simulink model "Odometry"  (R2023b)
settings: Solver=FixedStepDiscrete  StartTime=0.0  StopTime=inf  FixedStep=t_sample_fast  RelTol=1e-3
settings Model: Creator=FIRSTMentor  LastModifiedBy=ander
settings OptimizationCC: DefaultParameterBehavior=Inlined  StrengthReduction=on  PassReuseOutputArgsAs=Individual arguments  ZeroExternalMemoryAtStartup=off  ZeroInternalMemoryAtStartup=off  OptimizeBlockOrder=speed  OptimizationPriority=Speed  OptimizationCustomize=off  MultiThreadedLoops=on  EfficientTunableParamExpr=on
settings DebuggingCC: MergeDetectMultiDrivingBlocksExec=none  ParameterTunabilityLossMsg=error
settings HardwareCC: ProdBitPerPointer=32  ProdBitPerSizeT=32  ProdBitPerPtrDiffT=32  ProdLargestAtomicInteger=Long  ProdWordSize=32  ProdHWDeviceType=ARM Compatible->ARM 7
settings ModelReferenceCC: PropagateSignalLabelsOutOfModel=off
settings SFSimCC: MATLABDynamicMemAlloc=off
settings RTWCC: Description=Embedded Coder  SystemTargetFile=ert.tlc  GenCodeOnly=on  TemplateMakefile=ert_default_tmf  Toolchain=MinGW64 | gmake (64-bit Windows)
settings CodeAppCC: ForceParamTrailComments=on  IgnoreCustomStorageClasses=off  OperatorAnnotations=on  SimulinkDataObjDesc=on  SFDataObjDesc=on  InsertBlockDesc=on
settings ERTTargetCC: TargetLangStandard=C99 (ISO)  UtilityFuncGeneration=Shared location  SupportVariableSizeSignals=on  ParenthesesLevel=Maximum  InlinedParameterPlacement=NonHierarchical  ERTCustomFileTemplate=example_file_process.tlc

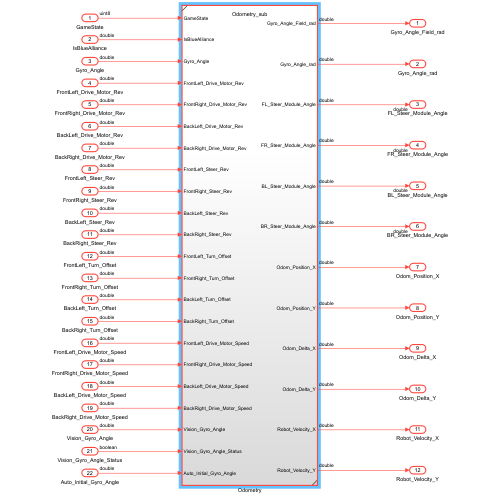
[thumbnail: Simulink's stored preview of the top-level diagram]
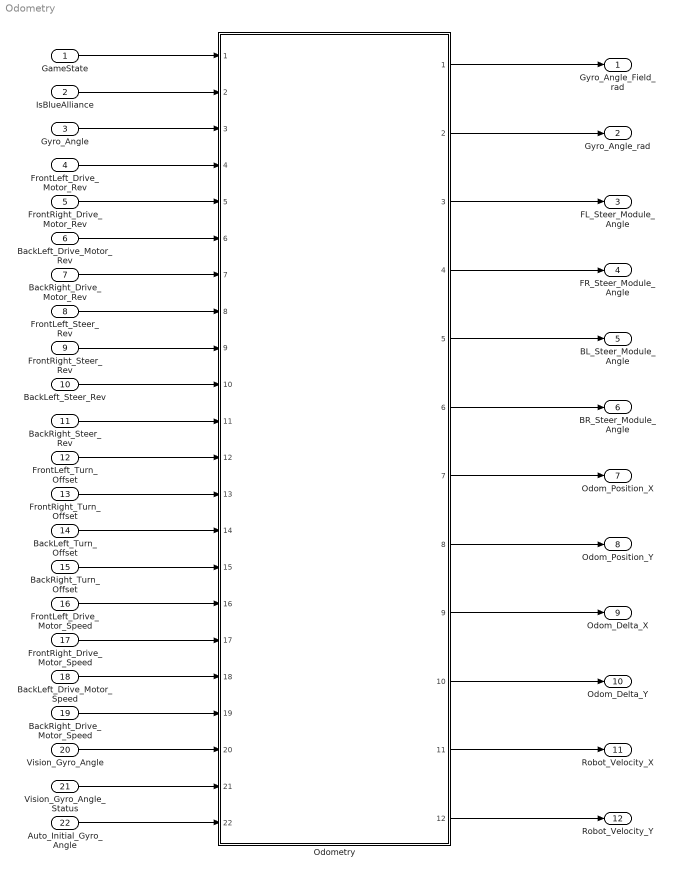
== system Odometry ==
  GameState : Inport
  IsBlueAlliance : Inport  Port=2
  Gyro_Angle : Inport  Port=3
  FrontLeft_Drive_Motor_Rev : Inport  Port=4
  FrontRight_Drive_Motor_Rev : Inport  Port=5
  BackLeft_Drive_Motor_Rev : Inport  Port=6
  BackRight_Drive_Motor_Rev : Inport  Port=7
  FrontLeft_Steer_Rev : Inport  Port=8
  FrontRight_Steer_Rev : Inport  Port=9
  BackLeft_Steer_Rev : Inport  Port=10
  BackRight_Steer_Rev : Inport  Port=11
  FrontLeft_Turn_Offset : Inport  Port=12
  FrontRight_Turn_Offset : Inport  Port=13
  BackLeft_Turn_Offset : Inport  Port=14
  BackRight_Turn_Offset : Inport  Port=15
  FrontLeft_Drive_Motor_Speed : Inport  Port=16
  FrontRight_Drive_Motor_Speed : Inport  Port=17
  BackLeft_Drive_Motor_Speed : Inport  Port=18
  BackRight_Drive_Motor_Speed : Inport  Port=19
  Vision_Gyro_Angle : Inport  Port=20
  Vision_Gyro_Angle_Status : Inport  Port=21
  Auto_Initial_Gyro_Angle : Inport  Port=22
  Odometry : Subsystem  ReferencedSubsystem=Odometry_sub
  Gyro_Angle_Field_rad : Outport
  Gyro_Angle_rad : Outport  Port=2
  FL_Steer_Module_Angle : Outport  Port=3  OutDataTypeStr=double  Unit=rad
  FR_Steer_Module_Angle : Outport  Port=4  OutDataTypeStr=double  Unit=rad
  BL_Steer_Module_Angle : Outport  Port=5  OutDataTypeStr=double  Unit=rad
  BR_Steer_Module_Angle : Outport  Port=6  OutDataTypeStr=double  Unit=rad
  Odom_Position_X : Outport  Port=7
  Odom_Position_Y : Outport  Port=8
  Odom_Delta_X : Outport  Port=9
  Odom_Delta_Y : Outport  Port=10
  Robot_Velocity_X : Outport  Port=11
  Robot_Velocity_Y : Outport  Port=12
  wires:
  FrontLeft_Drive_Motor_Rev/1 -> Odometry/4
  FrontRight_Drive_Motor_Rev/1 -> Odometry/5
  Gyro_Angle/1 -> Odometry/3
  BackLeft_Drive_Motor_Rev/1 -> Odometry/6
  IsBlueAlliance/1 -> Odometry/2
  BackRight_Drive_Motor_Rev/1 -> Odometry/7
  FrontLeft_Steer_Rev/1 -> Odometry/8
  FrontRight_Steer_Rev/1 -> Odometry/9
  BackLeft_Steer_Rev/1 -> Odometry/10
  BackRight_Steer_Rev/1 -> Odometry/11
  FrontLeft_Turn_Offset/1 -> Odometry/12
  FrontRight_Turn_Offset/1 -> Odometry/13
  BackLeft_Turn_Offset/1 -> Odometry/14
  BackRight_Turn_Offset/1 -> Odometry/15
  Odometry/1 -> Gyro_Angle_Field_rad/1
  Odometry/2 -> Gyro_Angle_rad/1
  Odometry/3 -> FL_Steer_Module_Angle/1
  Odometry/4 -> FR_Steer_Module_Angle/1
  Odometry/5 -> BL_Steer_Module_Angle/1
  Odometry/6 -> BR_Steer_Module_Angle/1
  Odometry/7 -> Odom_Position_X/1
  Odometry/8 -> Odom_Position_Y/1
  Odometry/9 -> Odom_Delta_X/1
  Odometry/10 -> Odom_Delta_Y/1
  FrontLeft_Drive_Motor_Speed/1 -> Odometry/16
  FrontRight_Drive_Motor_Speed/1 -> Odometry/17
  BackLeft_Drive_Motor_Speed/1 -> Odometry/18
  BackRight_Drive_Motor_Speed/1 -> Odometry/19
  Odometry/12 -> Robot_Velocity_Y/1
  Odometry/11 -> Robot_Velocity_X/1
  Vision_Gyro_Angle/1 -> Odometry/20
  Vision_Gyro_Angle_Status/1 -> Odometry/21
  GameState/1 -> Odometry/1
  Auto_Initial_Gyro_Angle/1 -> Odometry/22
